simulink model "Motor_moddel"  (R2026a)
settings: Solver=VariableStepAuto  MaxStep=0.001
values from neighbouring files (symbols this model uses):
  B = 0.15    [Motor_model_param.m]
  D = 3.323e-6    (= 3.323e-06)    [Motor_model_param.m]
  gear = 9.68    [Motor_model_param.m]
  J = 5.4619e-6    (= 5.4619e-06)    [Motor_model_param.m]
  Kb = Kt    (= 0.007956)    [Motor_model_param.m]
  Kp = 0.05    [Motor_model_param.m]
  Kpt = 5    [Motor_model_param.m]
  Kt = 0.007956    [Motor_model_param.m]
  L = 0.00380    (= 0.0038)    [Motor_model_param.m]
  R = 2.84    [Motor_model_param.m]
  taui_t = 0.2    [Motor_model_param.m]
  wrad = 0.03    [Motor_model_param.m]
settings Model: Creator=mariu  LastModifiedBy=mariu

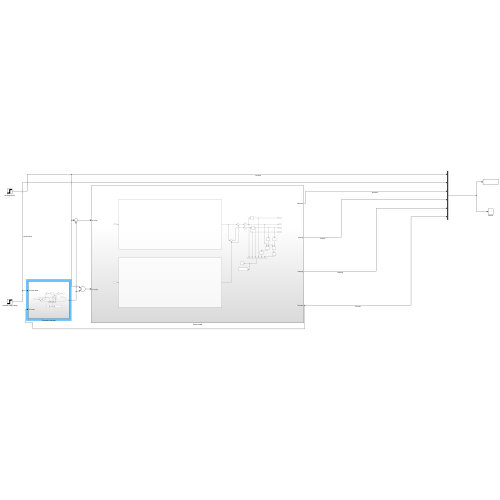
[thumbnail: Simulink's stored preview of the top-level diagram]
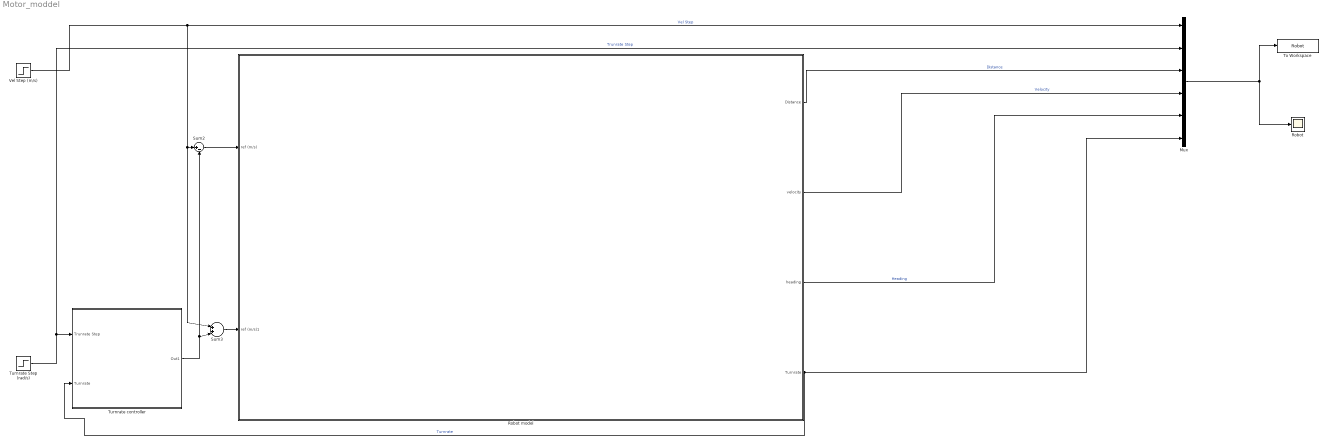
== system Motor_moddel ==
  Mux : Mux  Inputs=6
  Robot : Scope
      settings: ActiveDisplayYMinimum=-4.0353779215896068  ActiveDisplayYMaximum=4.8076313344836894
  Robot model : Subsystem
  Sum2 : Sum  Inputs=|+-
  Sum3 : Sum  Inputs=|++|
  To Workspace : ToWorkspace  VariableName=Robot  SaveFormat=Timeseries  SampleTime=-1
  Turnrate Step (rad/s) : Step  Time=0.5  SampleTime=0
  Turnrate controller : Subsystem
  Vel Step (m/s) : Step  Time=0.1  FinalValue=0.6  SampleTime=0
  wires:
  Robot model/1(Distance) -> Mux/3  "Distance"
  Robot model/2(velocity) -> Mux/4  "Velocity"
  Robot model/3(heading) -> Mux/5  "Heading"
  Robot model/4(Turnrate) -> Turnrate controller/2(Turnrate), Mux/6  "Turnrate"
  Vel Step (m/s)/1 -> Sum3/1, Sum2/1, Mux/1  "Vel Step"
  Turnrate Step (rad/s)/1 -> Turnrate controller/1(Trunrate Step), Mux/2  "Trunrate Step"
  Mux/1 -> To Workspace/1, Robot/1
  Sum2/1 -> Robot model/1(ref (m/s))
  Sum3/1 -> Robot model/2(ref (m/s)1)
  Turnrate controller/1(Out1) -> Sum2/2, Sum3/2

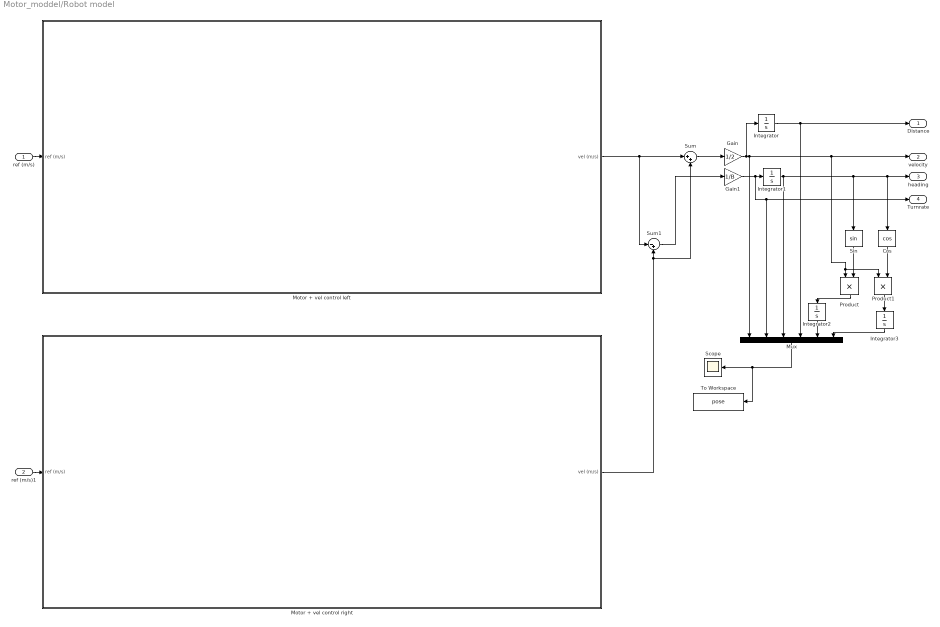
== system Motor_moddel/Robot model ==
  ref (m/s) : Inport
  ref (m/s)1 : Inport  Port=2
  Cos : Trigonometry  Operator=cos
  Gain : Gain  Gain=1/2
  Gain1 : Gain  Gain=1/B
  Integrator{,1..3} (4 alike) : Integrator
  Motor + vel control left : Subsystem
  Motor + vel control right : Subsystem
  Mux : Mux  Inputs=6
  Product : Product
  Product1 : Product
  Scope : Scope
      settings: ActiveDisplayYMinimum=-0.1149883215671369  ActiveDisplayYMaximum=0.30477624997481578
  Sin : Trigonometry
  Sum : Sum  Inputs=|++
  Sum1 : Sum  Inputs=|-+
  To Workspace : ToWorkspace  VariableName=pose  SaveFormat=Timeseries  SampleTime=-1
  Distance : Outport
  velocity : Outport  Port=2
  heading : Outport  Port=3
  Turnrate : Outport  Port=4
  wires:
  Integrator1/1 -> Mux/3, Sin/1, heading/1, Cos/1
  Motor + vel control left/1(vel (m/s)) -> Sum1/1, Sum/1
  Gain/1 -> Mux/1, velocity/1, Product1/1, Product/1, Integrator/1
  Gain1/1 -> Turnrate/1, Mux/2, Integrator1/1
  Integrator3/1 -> Mux/6
  Motor + vel control right/1(vel (m/s)) -> Sum/2, Sum1/2
  Product1/1 -> Integrator3/1
  Mux/1 -> To Workspace/1, Scope/1
  Sum/1 -> Gain/1
  Integrator/1 -> Distance/1, Mux/4
  Sin/1 -> Product/2
  Integrator2/1 -> Mux/5
  Sum1/1 -> Gain1/1
  Cos/1 -> Product1/2
  Product/1 -> Integrator2/1
  ref (m/s)1/1 -> Motor + vel control right/1(ref (m/s))
  ref (m/s)/1 -> Motor + vel control left/1(ref (m/s))

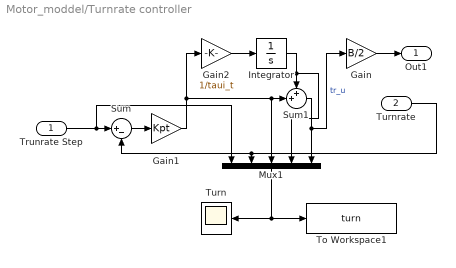
== system Motor_moddel/Turnrate controller ==
  Trunrate Step : Inport
  Turnrate : Inport  Port=2
  Gain : Gain  Gain=B/2
  Gain1 : Gain  Gain=Kpt
  Gain2 : Gain  Gain=1/taui_t
  Integrator : Integrator
  Mux1 : Mux  Inputs=5
  Sum : Sum  Inputs=|+-
  Sum1 : Sum  Inputs=++|
  To Workspace1 : ToWorkspace  VariableName=turn  SaveFormat=Timeseries  SampleTime=-1
  Turn : Scope
      settings: ActiveDisplayYMinimum=-3.2340238450026884  ActiveDisplayYMaximum=5.5625461017810185  DataLoggingVariableName=ScopeData2
  Out1 : Outport
  wires:
  Sum1/1 -> Mux1/5, Gain/1  "tr_u"
  Mux1/1 -> Turn/1, To Workspace1/1
  Gain1/1 -> Gain2/1, Mux1/3, Sum1/2
  Sum/1 -> Gain1/1
  Trunrate Step/1 -> Mux1/1, Sum/1
  Turnrate/1 -> Sum/2, Mux1/2
  Integrator/1 -> Mux1/4, Sum1/1
  Gain2/1 -> Integrator/1
  Gain/1 -> Out1/1

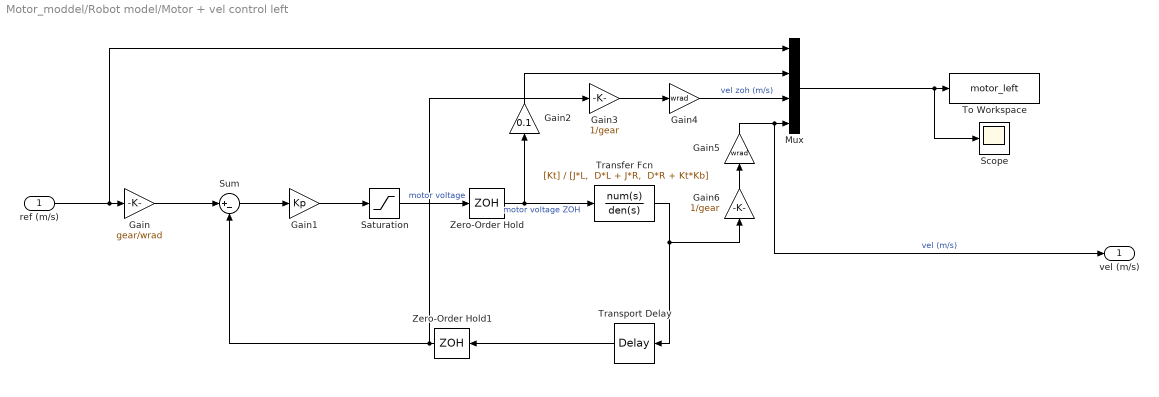
== system Motor_moddel/Robot model/Motor + vel control left ==
  ref (m/s) : Inport
  Gain : Gain  Gain=gear/wrad
  Gain1 : Gain  Gain=Kp
  Gain2 : Gain  Gain=0.1
  Gain3 : Gain  Gain=1/gear
  Gain4 : Gain  Gain=wrad
  Gain5 : Gain  Gain=wrad
  Gain6 : Gain  Gain=1/gear
  Mux : Mux
  Saturation : Saturate  UpperLimit=9  LowerLimit=-9
  Scope : Scope
      settings: ActiveDisplayYMinimum=-2.71992275563529  ActiveDisplayYMaximum=2.9624647860857189
  Sum : Sum  Inputs=|+-
  To Workspace : ToWorkspace  VariableName=motor_left  SaveFormat=Timeseries  SampleTime=-1
  Transfer Fcn : TransferFcn  Numerator=[Kt]  Denominator="[J*L,  D*L + J*R,  D*R + Kt*Kb]"
  Transport Delay : TransportDelay  DelayTime=0.01
  Zero-Order Hold : ZeroOrderHold  SampleTime=-1
  Zero-Order Hold1 : ZeroOrderHold  SampleTime=-1
  vel (m/s) : Outport
  wires:
  Gain5/1 -> vel (m/s)/1, Mux/4  "vel (m/s)"
  Zero-Order Hold/1 -> Transfer Fcn/1, Gain2/1  "motor voltage ZOH"
  Gain4/1 -> Mux/3  "vel zoh (m/s)"
  Mux/1 -> Scope/1, To Workspace/1
  Gain6/1 -> Gain5/1
  Gain1/1 -> Saturation/1
  Gain2/1 -> Mux/2
  Transfer Fcn/1 -> Gain6/1, Transport Delay/1
  Gain3/1 -> Gain4/1
  Zero-Order Hold1/1 -> Gain3/1, Sum/2
  ref (m/s)/1 -> Mux/1, Gain/1
  Transport Delay/1 -> Zero-Order Hold1/1
  Saturation/1 -> Zero-Order Hold/1  "motor voltage"
  Gain/1 -> Sum/1
  Sum/1 -> Gain1/1

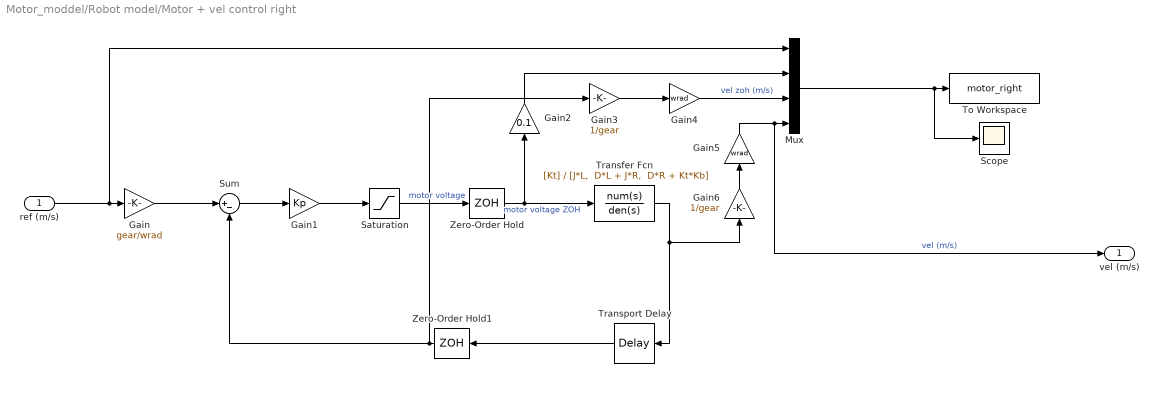
== system Motor_moddel/Robot model/Motor + vel control right ==
  ref (m/s) : Inport
  Gain : Gain  Gain=gear/wrad
  Gain1 : Gain  Gain=Kp
  Gain2 : Gain  Gain=0.1
  Gain3 : Gain  Gain=1/gear
  Gain4 : Gain  Gain=wrad
  Gain5 : Gain  Gain=wrad
  Gain6 : Gain  Gain=1/gear
  Mux : Mux
  Saturation : Saturate  UpperLimit=9  LowerLimit=-9
  Scope : Scope
  Sum : Sum  Inputs=|+-
  To Workspace : ToWorkspace  VariableName=motor_right  SaveFormat=Timeseries  SampleTime=-1
  Transfer Fcn : TransferFcn  Numerator=[Kt]  Denominator="[J*L,  D*L + J*R,  D*R + Kt*Kb]"
  Transport Delay : TransportDelay  DelayTime=0.01
  Zero-Order Hold : ZeroOrderHold  SampleTime=-1
  Zero-Order Hold1 : ZeroOrderHold  SampleTime=-1
  vel (m/s) : Outport
  wires:
  Gain5/1 -> vel (m/s)/1, Mux/4  "vel (m/s)"
  Zero-Order Hold/1 -> Transfer Fcn/1, Gain2/1  "motor voltage ZOH"
  Gain4/1 -> Mux/3  "vel zoh (m/s)"
  Mux/1 -> Scope/1, To Workspace/1
  Gain6/1 -> Gain5/1
  Gain1/1 -> Saturation/1
  Gain2/1 -> Mux/2
  Transfer Fcn/1 -> Gain6/1, Transport Delay/1
  Gain3/1 -> Gain4/1
  Zero-Order Hold1/1 -> Gain3/1, Sum/2
  ref (m/s)/1 -> Mux/1, Gain/1
  Transport Delay/1 -> Zero-Order Hold1/1
  Saturation/1 -> Zero-Order Hold/1  "motor voltage"
  Gain/1 -> Sum/1
  Sum/1 -> Gain1/1
